simulink model "hopper_6dof"  (R2026b)
settings: Solver=FixedStepAuto  StopTime=tgrid(end)  FixedStep=1e-3  RelTol=1e-5
undefined symbols (not defined in the file): cg_init, controller_start_time, fdir_params, fsw_latency, fsw_period, g, IN, K1flat, K1flat_lo, K2grid, Klqi, nav_dt, nav_g, nav_init, nav_Qc, nav_reset, OUT, p, sensor_params, Target_Trajectory, tgrid, u_hold_command, unom, VEH
libraries: fl_lib x43, nesl_utility x31, SimscapeFluids_lib x13, slpidlib x3, simulink_extras x2, commrandsrc3 x1, dspsrcs4 x1, matrix_library x1, aerolibutil x1
(part 1 of 6)
settings Model: DataDictionary=hopper_harness.sldd  Creator=asing  LastModifiedBy=asing
settings DebuggingCC: SignalInfNanChecking=warning
settings SimscapeCC: SimscapeUseEnergyAccounting=off

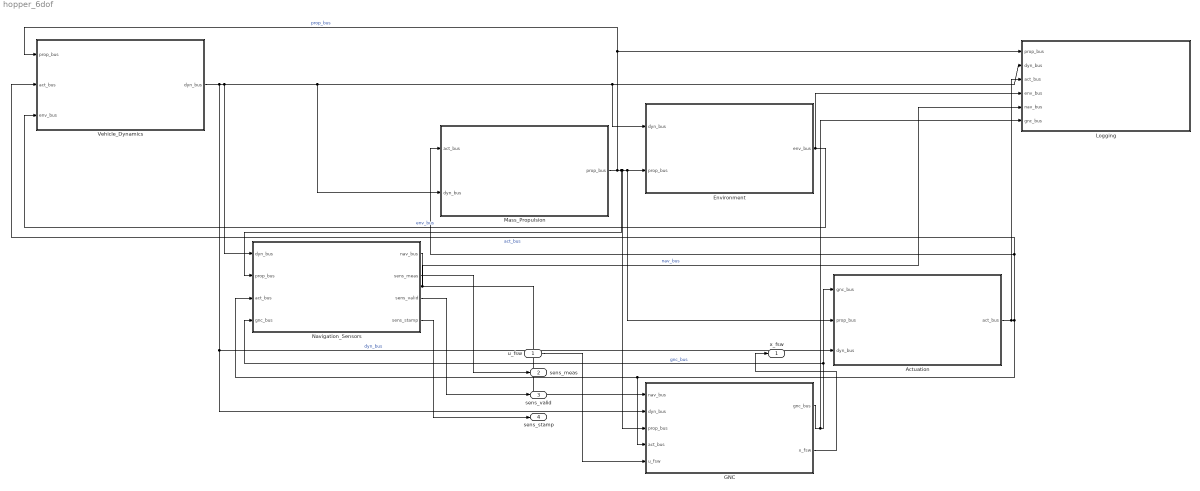
== system hopper_6dof ==
  u_fsw : Inport  OutDataTypeStr=double  PortDimensions=4  Interpolate=off
  Actuation : Subsystem
  Environment : Subsystem
  GNC : Subsystem
  Logging : Subsystem
  Mass_Propulsion : Subsystem
  Navigation_Sensors : Subsystem
  Vehicle_Dynamics : Subsystem
  x_fsw : Outport
  sens_meas : Outport  Port=2
  sens_valid : Outport  Port=3
  sens_stamp : Outport  Port=4
  wires:
  Vehicle_Dynamics/1(dyn_bus) -> GNC/2(dyn_bus), Actuation/3(dyn_bus), Environment/1(dyn_bus), Logging/2(dyn_bus), Mass_Propulsion/2(dyn_bus), Navigation_Sensors/1(dyn_bus)  "dyn_bus"
  GNC/1(gnc_bus) -> Navigation_Sensors/4(gnc_bus), Actuation/1(gnc_bus), Logging/6(gnc_bus)  "gnc_bus"
  Navigation_Sensors/1(nav_bus) -> GNC/1(nav_bus), Logging/5(nav_bus)  "nav_bus"
  Environment/1(env_bus) -> Vehicle_Dynamics/3(env_bus), Logging/4(env_bus)  "env_bus"
  Mass_Propulsion/1(prop_bus) -> Actuation/2(prop_bus), Environment/2(prop_bus), GNC/3(prop_bus), Navigation_Sensors/2(prop_bus), Logging/1(prop_bus), Vehicle_Dynamics/1(prop_bus)  "prop_bus"
  Actuation/1(act_bus) -> GNC/4(act_bus), Navigation_Sensors/3(act_bus), Mass_Propulsion/1(act_bus), Vehicle_Dynamics/2(act_bus), Logging/3(act_bus)  "act_bus"
  u_fsw/1 -> GNC/5(u_fsw)
  GNC/2(x_fsw) -> x_fsw/1
  Navigation_Sensors/2(sens_meas) -> sens_meas/1
  Navigation_Sensors/3(sens_valid) -> sens_valid/1
  Navigation_Sensors/4(sens_stamp) -> sens_stamp/1

== system hopper_6dof/Actuation ==
  u_cmd : Inport  PortName=gnc_bus  Element=u_cmd
  thrust : Inport  Port=2  PortName=prop_bus  Element=thrust
  cg : Inport  Port=2  PortName=prop_bus  Element=cg
  engine_cg : Inport  Port=2  PortName=prop_bus  Element=engine_cg
  mass : Inport  Port=2  PortName=prop_bus  Element=mass
  g_body : Inport  Port=3  PortName=dyn_bus  Element=g_body
  Actuators_TVC_RCS : Subsystem  ReferencedSubsystem=Actuators_TVC_RCS
  Demux : Demux
  IC : InitialCondition  Value=VEH.mass.wet*g
  Product : Product
  Quantizer : Quantizer  QuantizationInterval=IN.throttle_valve.resolution
  Rate Limiter1 : RateLimiter  RisingSlewLimit=IN.throttle_valve.rate_limit  FallingSlewLimit=-IN.throttle_valve.rate_limit  SampleTimeMode=inherited
  Saturation2 : Saturate  UpperLimit=IN.propulsion.nominal_thrust * IN.propulsion.throttle_range(2)  LowerLimit=IN.propulsion.nominal_thrust * IN.propulsion.throttle_range(1)
  Transport Delay2 : TransportDelay  DelayTime=IN.throttle_valve_latency
  Warmup_Control_Gate : Subsystem
  force : Outport  PortName=act_bus  Element=force
  moment : Outport  PortName=act_bus  Element=moment
  tvc_pitch : Outport  PortName=act_bus  Element=tvc_pitch
  tvc_yaw : Outport  PortName=act_bus  Element=tvc_yaw
  thrust_req : Outport  PortName=act_bus  Element=thrust_req
  thrust_cmd : Outport  PortName=act_bus  Element=thrust_cmd
  wires:
  IC/1 -> thrust_req/1, Saturation2/1
  Product/1 -> Actuators_TVC_RCS/5
  thrust/1 -> Actuators_TVC_RCS/1
  Demux/4 -> Actuators_TVC_RCS/4
  Demux/3 -> Actuators_TVC_RCS/3
  Demux/2 -> Actuators_TVC_RCS/2
  Demux/1 -> IC/1
  cg/1 -> Actuators_TVC_RCS/6
  engine_cg/1 -> Actuators_TVC_RCS/7
  Actuators_TVC_RCS/2 -> moment/1
  g_body/1 -> Product/1
  mass/1 -> Product/2, Actuators_TVC_RCS/8
  Actuators_TVC_RCS/1 -> force/1
  Actuators_TVC_RCS/3 -> tvc_pitch/1
  Actuators_TVC_RCS/4 -> tvc_yaw/1
  u_cmd/1 -> Warmup_Control_Gate/1(In1)
  Warmup_Control_Gate/1(Out1) -> Demux/1
  Quantizer/1 -> thrust_cmd/1
  Transport Delay2/1 -> Quantizer/1
  Saturation2/1 -> Rate Limiter1/1
  Rate Limiter1/1 -> Transport Delay2/1

== system hopper_6dof/Environment ==
  vel_ned : Inport  PortName=dyn_bus  Element=vel_ned
  dcm_be : Inport  PortName=dyn_bus  Element=dcm_be
  cg : Inport  Port=2  PortName=prop_bus  Element=cg
  Bernoulli Binary Generator : commrandsrc3/Bernoulli Binary Generator  ProbabilityOfZero=0.95  SeedSource=Parameter  Seed=0  SampleTime=0.1  SamplesPerFrame=1  OutputDataType=double  SimulateUsing=Interpreted execution
  MatrixMultiply1 : Product  Multiplication=Matrix(*)
  MatrixMultiply2 : Product  Multiplication=Matrix(*)
  Product1 : Product
  Random Source : dspsrcs4/Random Source  SrcType=Gaussian  MinVal=0  MaxVal=1  MeanVal=0  VarVal=IN.vehicle.disturbance.roll_torque_var  RepMode=Specify seed  rawSeed=1  IsInherit=off  SampTime=1  SampFrame=1  OutComplex=Real  DataType=double  SimulateUsing=Interpreted execution
  Wind_Forces : Subsystem  ReferencedSubsystem=Wind_Forces
  wind_force : Outport  PortName=env_bus  Element=wind_force
  wind_moment : Outport  PortName=env_bus  Element=wind_moment
  roll_dist : Outport  PortName=env_bus  Element=roll_dist
  wires:
  Bernoulli Binary Generator/1 -> Product1/1
  Random Source/1 -> Product1/2
  Wind_Forces/1 -> MatrixMultiply1/2
  Wind_Forces/2 -> MatrixMultiply2/2
  Product1/1 -> roll_dist/1
  cg/1 -> Wind_Forces/2
  vel_ned/1 -> Wind_Forces/1
  dcm_be/1 -> MatrixMultiply1/1, MatrixMultiply2/1, Wind_Forces/3
  MatrixMultiply1/1 -> wind_force/1
  MatrixMultiply2/1 -> wind_moment/1

== system hopper_6dof/GNC ==
  x_nav : Inport  PortName=nav_bus  Element=x_nav
  dcm_nav : Inport  PortName=nav_bus  Element=dcm_nav
  meas : Inport  PortName=nav_bus  Element=meas
  valid : Inport  PortName=nav_bus  Element=valid
  stamp : Inport  PortName=nav_bus  Element=stamp
  x_filt : Inport  PortName=nav_bus  Element=x_filt
  p_cov : Inport  PortName=nav_bus  Element=p_cov
  nav_diag : Inport  PortName=nav_bus  Element=nav_diag
  shadow : Inport  PortName=nav_bus  Element=shadow
  x_vert : Inport  PortName=nav_bus  Element=x_vert
  f_body : Inport  Port=2  PortName=dyn_bus  Element=f_body
  thrust : Inport  Port=3  PortName=prop_bus  Element=thrust
  mass : Inport  Port=3  PortName=prop_bus  Element=mass
  tvc_pitch : Inport  Port=4  PortName=act_bus  Element=tvc_pitch
  tvc_yaw : Inport  Port=4  PortName=act_bus  Element=tvc_yaw
  moment : Inport  Port=4  PortName=act_bus  Element=moment
  u_fsw : Inport  Port=5
  Actuator_Faults : Subsystem  Variant=on
  Controller : Subsystem  Variant=on  PropagateVariantConditions=on
  FDIR : Subsystem  Variant=on
  nav_mask : Outport  PortName=gnc_bus  Element=nav_mask
  nav_r_scale : Outport  PortName=gnc_bus  Element=nav_r_scale
  u_cmd : Outport  PortName=gnc_bus  Element=u_cmd
  x_fsw : Outport  Port=2
  wires:
  tvc_yaw/1 -> FDIR/7(tvc_yaw)
  x_nav/1 -> FDIR/2(x), Controller/1(x)
  f_body/1 -> FDIR/3(f_b)
  FDIR/3(nav_r_scale) -> nav_r_scale/1  "FDIR_nav_r_scale"
  Controller/1(u) -> FDIR/1(u_nom)
  dcm_nav/1 -> FDIR/4(dcm_be)
  meas/1 -> FDIR/10(meas)
  thrust/1 -> FDIR/5(thrust)
  tvc_pitch/1 -> FDIR/6(tvc_pitch)
  moment/1 -> FDIR/8(Mxyz)
  mass/1 -> FDIR/9(mass)
  valid/1 -> FDIR/11(valid)
  stamp/1 -> FDIR/12(stamp)
  x_filt/1 -> FDIR/13(xn)
  p_cov/1 -> FDIR/14(P)
  nav_diag/1 -> FDIR/15(diag)
  shadow/1 -> FDIR/16(shadow)
  x_vert/1 -> FDIR/17(x_vert)
  FDIR/2(nav_mask) -> nav_mask/1  "FDIR_nav_mask"
  FDIR/1(u) -> Actuator_Faults/1(u_in)
  Actuator_Faults/1(u) -> u_cmd/1
  u_fsw/1 -> Controller/2(u_fsw)
  Controller/2(x_fsw) -> x_fsw/1

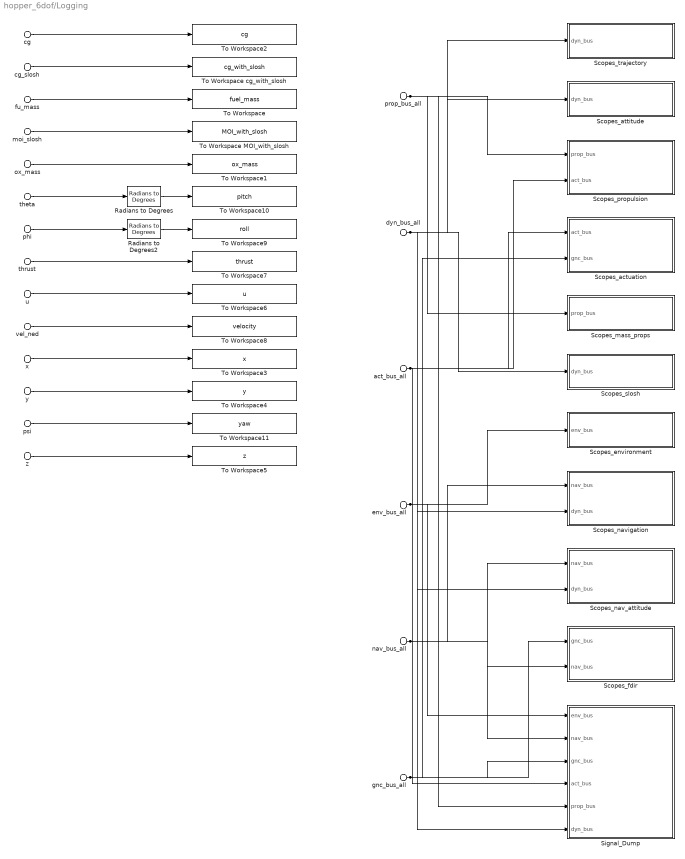
== system hopper_6dof/Logging ==
  prop_bus_all : Inport  PortName=prop_bus
  fu_mass : Inport  PortName=prop_bus  Element=fu_mass
  ox_mass : Inport  PortName=prop_bus  Element=ox_mass
  cg : Inport  PortName=prop_bus  Element=cg
  thrust : Inport  PortName=prop_bus  Element=thrust
  moi_slosh : Inport  PortName=prop_bus  Element=moi_slosh
  cg_slosh : Inport  PortName=prop_bus  Element=cg_slosh
  dyn_bus_all : Inport  Port=2  PortName=dyn_bus
  x : Inport  Port=2  PortName=dyn_bus  Element=x
  y : Inport  Port=2  PortName=dyn_bus  Element=y
  z : Inport  Port=2  PortName=dyn_bus  Element=z
  u : Inport  Port=2  PortName=dyn_bus  Element=u
  vel_ned : Inport  Port=2  PortName=dyn_bus  Element=vel_ned
  psi : Inport  Port=2  PortName=dyn_bus  Element=psi
  theta : Inport  Port=2  PortName=dyn_bus  Element=theta
  phi : Inport  Port=2  PortName=dyn_bus  Element=phi
  act_bus_all : Inport  Port=3  PortName=act_bus
  env_bus_all : Inport  Port=4  PortName=env_bus
  nav_bus_all : Inport  Port=5  PortName=nav_bus
  gnc_bus_all : Inport  Port=6  PortName=gnc_bus
  Radians to Degrees : simulink_extras/Transformations/Radians to Degrees
  Radians to Degrees2 : simulink_extras/Transformations/Radians to Degrees
  Scopes_actuation : Subsystem  Variant=on  EmptyChoice=on
  Scopes_attitude : Subsystem  Variant=on  EmptyChoice=on
  Scopes_environment : Subsystem  Variant=on  EmptyChoice=on
  Scopes_fdir : Subsystem  Variant=on  EmptyChoice=on
  Scopes_mass_props : Subsystem  Variant=on  EmptyChoice=on
  Scopes_nav_attitude : Subsystem  Variant=on  EmptyChoice=on
  Scopes_navigation : Subsystem  Variant=on  EmptyChoice=on
  Scopes_propulsion : Subsystem  Variant=on  EmptyChoice=on
  Scopes_slosh : Subsystem  Variant=on  EmptyChoice=on
  Scopes_trajectory : Subsystem  Variant=on  EmptyChoice=on
  Signal_Dump : Subsystem  Variant=on  EmptyChoice=on
  To Workspace : ToWorkspace  VariableName=fuel_mass  SaveFormat=Timeseries  SampleTime=-1
  To Workspace MOI_with_slosh : ToWorkspace  VariableName=MOI_with_slosh  SaveFormat=Timeseries  SampleTime=-1
  To Workspace cg_with_slosh : ToWorkspace  VariableName=cg_with_slosh  SaveFormat=Timeseries  SampleTime=-1
  To Workspace1 : ToWorkspace  VariableName=ox_mass  SaveFormat=Timeseries  SampleTime=-1
  To Workspace10 : ToWorkspace  VariableName=pitch  SaveFormat=Timeseries  SampleTime=-1
  To Workspace11 : ToWorkspace  VariableName=yaw  SaveFormat=Timeseries  SampleTime=-1
  To Workspace2 : ToWorkspace  VariableName=cg  SaveFormat=Timeseries  SampleTime=-1
  To Workspace3 : ToWorkspace  VariableName=x  SaveFormat=Timeseries  SampleTime=-1
  To Workspace4 : ToWorkspace  VariableName=y  SaveFormat=Timeseries  SampleTime=-1
  To Workspace5 : ToWorkspace  VariableName=z  SaveFormat=Timeseries  SampleTime=-1
  To Workspace6 : ToWorkspace  VariableName=u  SaveFormat=Timeseries  SampleTime=-1
  To Workspace7 : ToWorkspace  VariableName=thrust  SaveFormat=Timeseries  SampleTime=-1
  To Workspace8 : ToWorkspace  VariableName=velocity  SaveFormat=Timeseries  SampleTime=-1
  To Workspace9 : ToWorkspace  VariableName=roll  SaveFormat=Timeseries  SampleTime=-1
  wires:
  u/1 -> To Workspace6/1
  vel_ned/1 -> To Workspace8/1
  thrust/1 -> To Workspace7/1
  phi/1 -> Radians to Degrees2/1
  moi_slosh/1 -> To Workspace MOI_with_slosh/1
  cg_slosh/1 -> To Workspace cg_with_slosh/1
  cg/1 -> To Workspace2/1
  theta/1 -> Radians to Degrees/1
  psi/1 -> To Workspace11/1
  Radians to Degrees2/1 -> To Workspace9/1
  ox_mass/1 -> To Workspace1/1
  fu_mass/1 -> To Workspace/1
  Radians to Degrees/1 -> To Workspace10/1
  x/1 -> To Workspace3/1
  y/1 -> To Workspace4/1
  z/1 -> To Workspace5/1
  dyn_bus_all/1 -> Scopes_trajectory/1(dyn_bus), Scopes_attitude/1(dyn_bus), Scopes_slosh/1(dyn_bus), Scopes_navigation/2(dyn_bus), Scopes_nav_attitude/2(dyn_bus), Signal_Dump/6(dyn_bus)
  prop_bus_all/1 -> Scopes_propulsion/1(prop_bus), Scopes_mass_props/1(prop_bus), Signal_Dump/5(prop_bus)
  act_bus_all/1 -> Scopes_propulsion/2(act_bus), Scopes_actuation/1(act_bus), Signal_Dump/4(act_bus)
  gnc_bus_all/1 -> Scopes_actuation/2(gnc_bus), Scopes_fdir/1(gnc_bus), Signal_Dump/3(gnc_bus)
  env_bus_all/1 -> Scopes_environment/1(env_bus), Signal_Dump/1(env_bus)
  nav_bus_all/1 -> Scopes_navigation/1(nav_bus), Scopes_nav_attitude/1(nav_bus), Scopes_fdir/2(nav_bus), Signal_Dump/2(nav_bus)

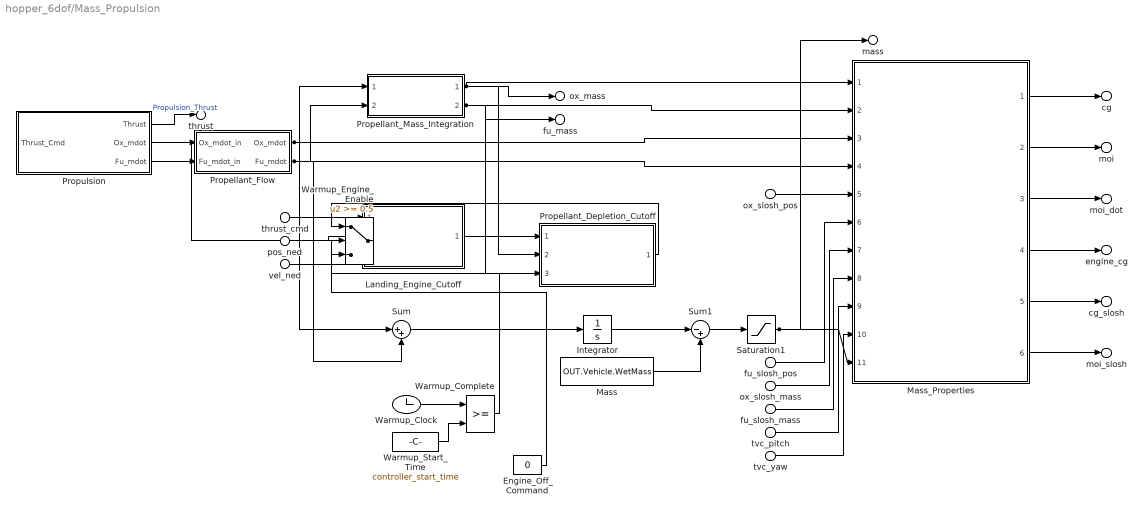
== system hopper_6dof/Mass_Propulsion ==
  thrust_cmd : Inport  PortName=act_bus  Element=thrust_cmd
  tvc_pitch : Inport  PortName=act_bus  Element=tvc_pitch
  tvc_yaw : Inport  PortName=act_bus  Element=tvc_yaw
  pos_ned : Inport  Port=2  PortName=dyn_bus  Element=pos_ned
  vel_ned : Inport  Port=2  PortName=dyn_bus  Element=vel_ned
  ox_slosh_pos : Inport  Port=2  PortName=dyn_bus  Element=ox_slosh_pos
  fu_slosh_pos : Inport  Port=2  PortName=dyn_bus  Element=fu_slosh_pos
  ox_slosh_mass : Inport  Port=2  PortName=dyn_bus  Element=ox_slosh_mass
  fu_slosh_mass : Inport  Port=2  PortName=dyn_bus  Element=fu_slosh_mass
  Engine_Off_Command : Constant  Value=0
  Integrator : Integrator
  Landing_Engine_Cutoff : Subsystem  ReferencedSubsystem=Landing_Engine_Cutoff
  Mass : Constant  Value=OUT.Vehicle.WetMass
  Mass_Properties : Subsystem  ReferencedSubsystem=Mass_Properties
  Propellant_Depletion_Cutoff : Subsystem  ReferencedSubsystem=Propellant_Depletion_Cutoff
  Propellant_Flow : Subsystem  Variant=on
  Propellant_Mass_Integration : Subsystem  ReferencedSubsystem=Propellant_Mass_Integration
  Propulsion : Subsystem  Variant=on
  Saturation1 : Saturate  UpperLimit=OUT.Vehicle.WetMass  LowerLimit=OUT.Vehicle.DryMass
  Sum : Sum  Inputs=|++
  Sum1 : Sum  Inputs=|-+
  Warmup_Clock : Clock
  Warmup_Complete : RelationalOperator  OutDataTypeStr=boolean  RndMeth=Simplest  InputSameDT=off
  Warmup_Engine_Enable : Switch  Threshold=0.5  SaturateOnIntegerOverflow=off  InputSameDT=off
  Warmup_Start_Time : Constant  Value=controller_start_time
  thrust : Outport  PortName=prop_bus  Element=thrust
  ox_mass : Outport  PortName=prop_bus  Element=ox_mass
  fu_mass : Outport  PortName=prop_bus  Element=fu_mass
  cg : Outport  PortName=prop_bus  Element=cg
  moi : Outport  PortName=prop_bus  Element=moi
  moi_dot : Outport  PortName=prop_bus  Element=moi_dot
  engine_cg : Outport  PortName=prop_bus  Element=engine_cg
  cg_slosh : Outport  PortName=prop_bus  Element=cg_slosh
  moi_slosh : Outport  PortName=prop_bus  Element=moi_slosh
  mass : Outport  PortName=prop_bus  Element=mass
  wires:
  Propulsion/1(Thrust) -> thrust/1  "Propulsion_Thrust"
  Propulsion/3(Fu_mdot) -> Propellant_Flow/2(Fu_mdot_in)
  Propellant_Mass_Integration/2 -> Mass_Properties/2, Propellant_Depletion_Cutoff/3, fu_mass/1
  Propellant_Mass_Integration/1 -> Mass_Properties/1, Propellant_Depletion_Cutoff/2, ox_mass/1
  Propulsion/2(Ox_mdot) -> Propellant_Flow/1(Ox_mdot_in)
  tvc_pitch/1 -> Mass_Properties/9
  ox_slosh_mass/1 -> Mass_Properties/7
  Propellant_Flow/1(Ox_mdot) -> Propellant_Mass_Integration/1, Mass_Properties/3, Sum/1
  Propellant_Flow/2(Fu_mdot) -> Sum/2, Mass_Properties/4, Propellant_Mass_Integration/2
  Mass_Properties/4 -> engine_cg/1
  Mass_Properties/3 -> moi_dot/1
  vel_ned/1 -> Landing_Engine_Cutoff/3
  pos_ned/1 -> Landing_Engine_Cutoff/2
  thrust_cmd/1 -> Landing_Engine_Cutoff/1
  Landing_Engine_Cutoff/1 -> Propellant_Depletion_Cutoff/1
  Sum/1 -> Integrator/1
  Integrator/1 -> Sum1/1
  Mass/1 -> Sum1/2
  Sum1/1 -> Saturation1/1
  ox_slosh_pos/1 -> Mass_Properties/5
  Saturation1/1 -> Mass_Properties/11, mass/1
  fu_slosh_pos/1 -> Mass_Properties/6
  tvc_yaw/1 -> Mass_Properties/10
  fu_slosh_mass/1 -> Mass_Properties/8
  Mass_Properties/2 -> moi/1
  Mass_Properties/1 -> cg/1
  Mass_Properties/6 -> moi_slosh/1
  Mass_Properties/5 -> cg_slosh/1
  Warmup_Clock/1 -> Warmup_Complete/1
  Warmup_Start_Time/1 -> Warmup_Complete/2
  Propellant_Depletion_Cutoff/1 -> Warmup_Engine_Enable/1
  Warmup_Complete/1 -> Warmup_Engine_Enable/2
  Engine_Off_Command/1 -> Warmup_Engine_Enable/3
  Warmup_Engine_Enable/1 -> Propulsion/1(Thrust_Cmd)

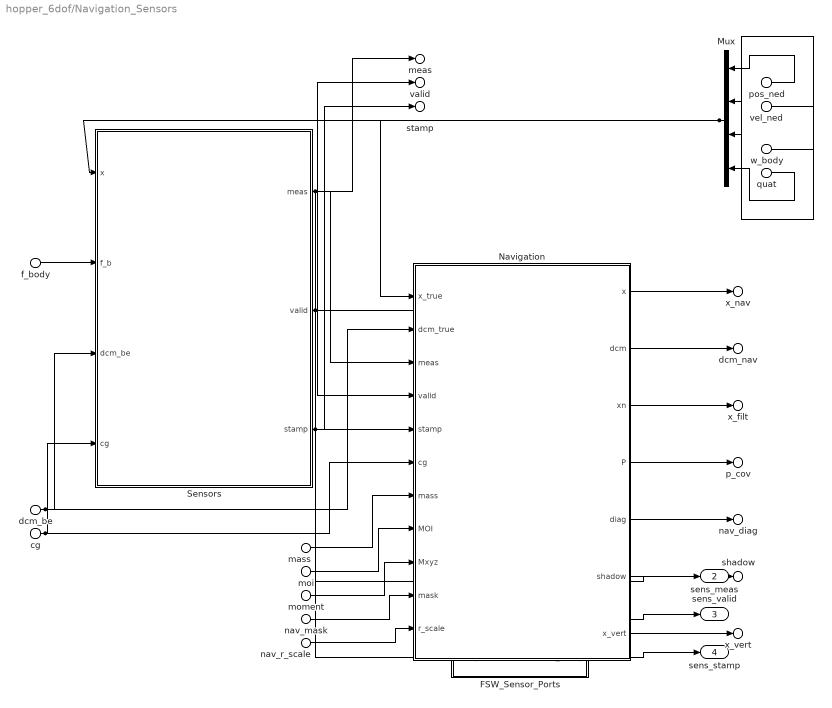
== system hopper_6dof/Navigation_Sensors ==
  f_body : Inport  PortName=dyn_bus  Element=f_body
  dcm_be : Inport  PortName=dyn_bus  Element=dcm_be
  pos_ned : Inport  PortName=dyn_bus  Element=pos_ned
  vel_ned : Inport  PortName=dyn_bus  Element=vel_ned
  w_body : Inport  PortName=dyn_bus  Element=w_body
  quat : Inport  PortName=dyn_bus  Element=quat
  cg : Inport  Port=2  PortName=prop_bus  Element=cg
  mass : Inport  Port=2  PortName=prop_bus  Element=mass
  moi : Inport  Port=2  PortName=prop_bus  Element=moi
  moment : Inport  Port=3  PortName=act_bus  Element=moment
  nav_mask : Inport  Port=4  PortName=gnc_bus  Element=nav_mask
  nav_r_scale : Inport  Port=4  PortName=gnc_bus  Element=nav_r_scale
  FSW_Sensor_Ports : Subsystem  Description=CONTROLLER=fsw only: the sensor model's meas/valid/stamp out to root sens_* ports for the flight-software plant. Built by tools/refactor/addFswSensorPorts.m.  Variant=on  EmptyChoice=on  PropagateVariantConditions=on
  Mux : Mux
  Navigation : Subsystem  Variant=on
  Sensors : Subsystem  Variant=on
  meas : Outport  PortName=nav_bus  Element=meas
  valid : Outport  PortName=nav_bus  Element=valid
  stamp : Outport  PortName=nav_bus  Element=stamp
  x_nav : Outport  PortName=nav_bus  Element=x_nav
  dcm_nav : Outport  PortName=nav_bus  Element=dcm_nav
  x_filt : Outport  PortName=nav_bus  Element=x_filt
  p_cov : Outport  PortName=nav_bus  Element=p_cov
  nav_diag : Outport  PortName=nav_bus  Element=nav_diag
  shadow : Outport  PortName=nav_bus  Element=shadow
  x_vert : Outport  PortName=nav_bus  Element=x_vert
  sens_meas : Outport  Port=2
  sens_valid : Outport  Port=3
  sens_stamp : Outport  Port=4
  wires:
  cg/1 -> Navigation/6(cg), Sensors/4(cg)
  f_body/1 -> Sensors/2(f_b)
  dcm_be/1 -> Navigation/2(dcm_true), Sensors/3(dcm_be)
  Navigation/2(dcm) -> dcm_nav/1
  Navigation/1(x) -> x_nav/1
  Sensors/1(meas) -> Navigation/3(meas), meas/1, FSW_Sensor_Ports/1(meas)
  Sensors/2(valid) -> valid/1, Navigation/4(valid), FSW_Sensor_Ports/2(valid)
  Sensors/3(stamp) -> Navigation/5(stamp), stamp/1, FSW_Sensor_Ports/3(stamp)
  mass/1 -> Navigation/7(mass)
  moi/1 -> Navigation/8(MOI)
  moment/1 -> Navigation/9(Mxyz)
  nav_mask/1 -> Navigation/10(mask)
  nav_r_scale/1 -> Navigation/11(r_scale)
  Navigation/4(P) -> p_cov/1
  Navigation/3(xn) -> x_filt/1
  vel_ned/1 -> Mux/2
  Navigation/6(shadow) -> shadow/1
  Navigation/5(diag) -> nav_diag/1
  Navigation/7(x_vert) -> x_vert/1
  Mux/1 -> Sensors/1(x), Navigation/1(x_true)
  pos_ned/1 -> Mux/1
  w_body/1 -> Mux/3
  quat/1 -> Mux/4
  FSW_Sensor_Ports/1(sens_meas) -> sens_meas/1
  FSW_Sensor_Ports/2(sens_valid) -> sens_valid/1
  FSW_Sensor_Ports/3(sens_stamp) -> sens_stamp/1

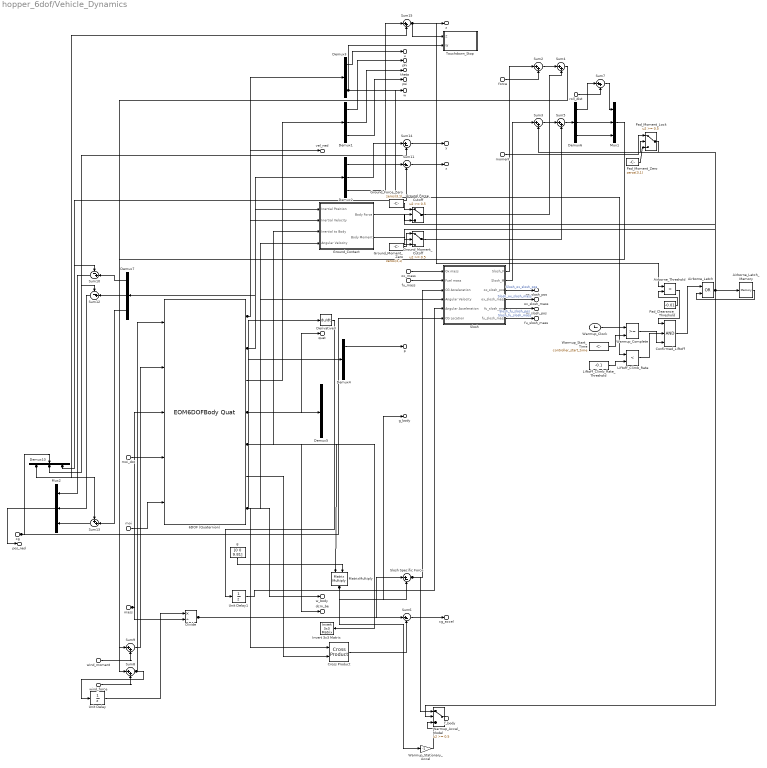
== system hopper_6dof/Vehicle_Dynamics ==
  mass : Inport  PortName=prop_bus  Element=mass
  moi_dot : Inport  PortName=prop_bus  Element=moi_dot
  moi : Inport  PortName=prop_bus  Element=moi
  ox_mass : Inport  PortName=prop_bus  Element=ox_mass
  fu_mass : Inport  PortName=prop_bus  Element=fu_mass
  cg : Inport  PortName=prop_bus  Element=cg
  force : Inport  Port=2  PortName=act_bus  Element=force
  moment : Inport  Port=2  PortName=act_bus  Element=moment
  roll_dist : Inport  Port=3  PortName=env_bus  Element=roll_dist
  wind_force : Inport  Port=3  PortName=env_bus  Element=wind_force
  wind_moment : Inport  Port=3  PortName=env_bus  Element=wind_moment
  6DOF (Quaternion) : EOM6DOFBodyQuat  mtype=Custom Variable  xme_0=[0 0 -cg_init]  eul_0=[0 pi/2 0]
  Airborne_Latch : Logic  Operator=OR  AllPortsSameDT=off  OutDataTypeStr=boolean
  Airborne_Latch_Memory : Memory
  Airborne_Threshold : RelationalOperator  Operator=<  OutDataTypeStr=boolean  RndMeth=Simplest  InputSameDT=off
  Confirmed_Liftoff : Logic  Inputs=3  AllPortsSameDT=off  OutDataTypeStr=boolean
  Cross Product : matrix_library/Cross Product
  Demux{1..4,6..7,10} (7 alike) : Demux  Outputs=3
  Demux5 : Demux
  Derivative3 : Derivative  CoefficientInTFapproximation=3
  Divide : Product  Inputs=*/
  Ground_Contact : Subsystem  Variant=on
  Ground_Force_Cutoff : Switch  Threshold=0.5  SaturateOnIntegerOverflow=off  InputSameDT=off
  Ground_Force_Zero : Constant  Value=zeros(3,1)
  Ground_Moment_Cutoff : Switch  Threshold=0.5  SaturateOnIntegerOverflow=off  InputSameDT=off
  Ground_Moment_Zero : Constant  Value=zeros(3,1)
  Invert 3x3 Matrix : aerolibutil/Invert  3x3 Matrix
  Liftoff_Climb_Rate : RelationalOperator  Operator=<  OutDataTypeStr=boolean  RndMeth=Simplest  InputSameDT=off
  Liftoff_Climb_Rate_Threshold : Constant  Value=-0.1
  MatrixMultiply : Product  Multiplication=Matrix(*)
  Mux1 : Mux  Inputs=3
  Mux2 : Mux  Inputs=3
  Pad_Clearance_Threshold : Constant  Value=-0.01
  Pad_Moment_Lock : Switch  Threshold=0.5  SaturateOnIntegerOverflow=off  InputSameDT=off
  Pad_Moment_Zero : Constant  Value=zeros(3,1)
  Slosh : Subsystem  Variant=on
  Slosh Specific Force : Sum  Description=(F_total/m) - g_body = non-gravitational specific force at the CG; drives the slosh pendulums.  Inputs=|+-
  Sum10 : Sum  Inputs=-+|
  Sum11 : Sum  Inputs=|+-
  Sum12 : Sum  Inputs=-+|
  Sum13 : Sum  Inputs=++|
  Sum14 : Sum  Inputs=|+-
  Sum{2..5,7..9,15} (8 alike) : Sum  Inputs=|++
  Sum6 : Sum  Inputs=|+-
  Touchdown_Stop : Subsystem  Description=Stops the run at the first descending ground contact, except with CONTROLLER=fsw and GROUND=strut (the flight software's plant rests on its struts). Built by tools/refactor/gateTouchdownStop.m.  Variant=on  EmptyChoice=on
  Unit Delay : UnitDelay  SampleTime=-1
  Unit Delay1 : UnitDelay  SampleTime=-1
  Warmup_Accel_Model : Switch  Threshold=0.5  SaturateOnIntegerOverflow=off  InputSameDT=off
  Warmup_Clock : Clock
  Warmup_Complete : RelationalOperator  OutDataTypeStr=boolean  RndMeth=Simplest  InputSameDT=off
  Warmup_Start_Time : Constant  Value=controller_start_time
  Warmup_Stationary_Accel : Gain  Gain=-1
  g : Constant  Value=[0 0 9.81]
  vel_ned : Outport  PortName=dyn_bus  Element=vel_ned
  quat : Outport  PortName=dyn_bus  Element=quat
  dcm_be : Outport  PortName=dyn_bus  Element=dcm_be
  w_body : Outport  PortName=dyn_bus  Element=w_body
  ox_slosh_pos : Outport  PortName=dyn_bus  Element=ox_slosh_pos
  ox_slosh_mass : Outport  PortName=dyn_bus  Element=ox_slosh_mass
  fu_slosh_pos : Outport  PortName=dyn_bus  Element=fu_slosh_pos
  fu_slosh_mass : Outport  PortName=dyn_bus  Element=fu_slosh_mass
  f_body : Outport  PortName=dyn_bus  Element=f_body
  cg_accel : Outport  PortName=dyn_bus  Element=cg_accel
  x : Outport  PortName=dyn_bus  Element=x
  y : Outport  PortName=dyn_bus  Element=y
  z : Outport  PortName=dyn_bus  Element=z
  phi : Outport  PortName=dyn_bus  Element=phi
  theta : Outport  PortName=dyn_bus  Element=theta
  psi : Outport  PortName=dyn_bus  Element=psi
  u : Outport  PortName=dyn_bus  Element=u
  w : Outport  PortName=dyn_bus  Element=w
  p : Outport  PortName=dyn_bus  Element=p
  pos_ned : Outport  PortName=dyn_bus  Element=pos_ned
  g_body : Outport  PortName=dyn_bus  Element=g_body
  wires:
  cg/1 -> Demux10/1, Slosh/6(CG Location)
  Sum13/1 -> Mux2/3
  Demux10/3 -> Sum10/1, Sum11/2
  Demux10/2 -> Sum12/1, Sum14/2
  Demux10/1 -> Sum13/1, Sum15/2
  Mux2/1 -> pos_ned/1
  MatrixMultiply/1 -> Slosh Specific Force/2, g_body/1, Warmup_Stationary_Accel/1
  Sum10/1 -> Mux2/1
  Sum12/1 -> Mux2/2
  wind_moment/1 -> Sum9/2
  wind_force/1 -> Sum8/2
  Unit Delay/1 -> Divide/1
  Demux7/3 -> Sum13/2
  Demux7/1 -> Sum10/2
  Demux7/2 -> Sum12/2
  moi_dot/1 -> 6DOF (Quaternion)/4
  moi/1 -> 6DOF (Quaternion)/5
  mass/1 -> 6DOF (Quaternion)/3, Divide/2
  Derivative3/1 -> Unit Delay1/1
  Sum9/1 -> 6DOF (Quaternion)/2
  Sum8/1 -> Unit Delay/1, 6DOF (Quaternion)/1
  g/1 -> MatrixMultiply/2
  Demux1/3 -> psi/1
  Demux1/2 -> theta/1
  6DOF (Quaternion)/1 -> Ground_Contact/2(Inertial Velocity), Demux3/1, vel_ned/1
  Unit Delay1/1 -> Slosh/5(Angular Acceleration)
  6DOF (Quaternion)/2 -> Demux7/1, Ground_Contact/1(Inertial Position), Demux2/1
  6DOF (Quaternion)/3 -> Demux1/1
  6DOF (Quaternion)/4 -> quat/1, Demux5/1
  Demux6/1 -> Sum7/1
  6DOF (Quaternion)/5 -> Invert 3x3 Matrix/1, Ground_Contact/3(Inertial to Body), MatrixMultiply/1, dcm_be/1
  6DOF (Quaternion)/6 -> Cross Product/2
  6DOF (Quaternion)/7 -> Demux4/1, Slosh/4(Angular Velocity), Cross Product/1, Derivative3/1, Ground_Contact/4(Angular Velocity), w_body/1
  Divide/1 -> Slosh Specific Force/1, Sum6/1
  Demux3/1 -> u/1
  Demux3/3 -> w/1, Liftoff_Climb_Rate/1, Touchdown_Stop/2(W)
  Demux1/1 -> phi/1
  Demux2/2 -> Sum14/1
  Demux2/1 -> Sum11/1
  Demux2/3 -> Sum15/1
  Demux4/1 -> p/1
  Sum3/1 -> Sum5/1
  Slosh/1(Slosh_F) -> Sum2/1
  Cross Product/1 -> Sum6/2
  Sum15/1 -> z/1, Airborne_Threshold/1, Touchdown_Stop/1(Z)
  Sum14/1 -> y/1
  Sum11/1 -> x/1
  ox_mass/1 -> Slosh/1(Ox mass)
  fu_mass/1 -> Slosh/2(Fuel mass)
  Slosh Specific Force/1 -> Slosh/3(CG Acceleration), Warmup_Accel_Model/1
  Sum6/1 -> cg_accel/1
  force/1 -> Sum2/2
  Slosh/3(ox_slosh_pos) -> ox_slosh_pos/1  "Slosh_ox_slosh_pos"
  Slosh/2(Slosh_M) -> Sum3/1
  Sum4/1 -> Sum8/1
  Slosh/5(fu_slosh_pos) -> fu_slosh_pos/1  "Slosh_fu_slosh_pos"
  Slosh/4(ox_slosh_mass) -> ox_slosh_mass/1  "Slosh_ox_slosh_mass"
  Slosh/6(fu_slosh_mass) -> fu_slosh_mass/1  "Slosh_fu_slosh_mass"
  Sum2/1 -> Sum4/1
  roll_dist/1 -> Sum7/2
  Demux6/2 -> Mux1/2
  Demux6/3 -> Mux1/3
  Sum7/1 -> Mux1/1
  Mux1/1 -> Sum9/1
  ? -> ?
  ? -> ?
  Ground_Force_Zero/1 -> Ground_Force_Cutoff/1
  Ground_Contact/1(Body Force) -> Ground_Force_Cutoff/3
  Ground_Force_Cutoff/1 -> Sum4/2
  Ground_Moment_Zero/1 -> Ground_Moment_Cutoff/1
  Ground_Contact/2(Body Moment) -> Ground_Moment_Cutoff/3
  Ground_Moment_Cutoff/1 -> Sum5/2
  Warmup_Stationary_Accel/1 -> Warmup_Accel_Model/3
  Warmup_Accel_Model/1 -> f_body/1
  Pad_Clearance_Threshold/1 -> Airborne_Threshold/2
  Airborne_Latch_Memory/1 -> Airborne_Latch/2
  Airborne_Latch/1 -> Airborne_Latch_Memory/1, Ground_Force_Cutoff/2, Ground_Moment_Cutoff/2, Warmup_Accel_Model/2, Pad_Moment_Lock/2
  Pad_Moment_Zero/1 -> Pad_Moment_Lock/3
  Warmup_Clock/1 -> Warmup_Complete/1
  Warmup_Start_Time/1 -> Warmup_Complete/2
  Liftoff_Climb_Rate_Threshold/1 -> Liftoff_Climb_Rate/2
  Airborne_Threshold/1 -> Confirmed_Liftoff/1
  Liftoff_Climb_Rate/1 -> Confirmed_Liftoff/2
  Warmup_Complete/1 -> Confirmed_Liftoff/3
  Confirmed_Liftoff/1 -> Airborne_Latch/1
  moment/1 -> Pad_Moment_Lock/1
  Pad_Moment_Lock/1 -> Sum3/2
  Sum5/1 -> Demux6/1

== system hopper_6dof/Actuation/Warmup_Control_Gate ==
  In1 : Inport
  After_Warmup : RelationalOperator  OutDataTypeStr=boolean  RndMeth=Simplest  InputSameDT=off
  Clock : Clock
  Hold_Command : Constant  Value=u_hold_command
  Select_Command : Switch  Threshold=0.5  SaturateOnIntegerOverflow=off  InputSameDT=off
  Start_Time : Constant  Value=controller_start_time
  Out1 : Outport
  wires:
  In1/1 -> Select_Command/1
  Clock/1 -> After_Warmup/1
  Start_Time/1 -> After_Warmup/2
  After_Warmup/1 -> Select_Command/2
  Hold_Command/1 -> Select_Command/3
  Select_Command/1 -> Out1/1

== system hopper_6dof/GNC/Actuator_Faults ==
  u_in : Inport
  Actuator_Faults_Off : Subsystem  VariantControl=VARIANT_FAULT_INJECTION == 1
  Actuator_Faults_On : Subsystem  VariantControl=VARIANT_FAULT_INJECTION == 2
  u : Outport

== system hopper_6dof/GNC/Controller ==
  x : Inport
  u_fsw : Inport  Port=2
  Controller_FSW : Subsystem  VariantControl=VARIANT_CONTROLLER == 5
  Controller_LQI : Subsystem  VariantControl=VARIANT_CONTROLLER == 2
  Controller_LQR_CTV_Tuning : Subsystem  VariantControl=VARIANT_CONTROLLER == 4
  Controller_LQR_Sched : Subsystem  VariantControl=VARIANT_CONTROLLER == 1
  Controller_LQR_Sched_Legacy : Subsystem  VariantControl=VARIANT_CONTROLLER == 3
  u : Outport
  x_fsw : Outport  Port=2

== system hopper_6dof/GNC/FDIR ==
  u_nom : Inport
  x : Inport  Port=2
  f_b : Inport  Port=3
  dcm_be : Inport  Port=4
  thrust : Inport  Port=5
  tvc_pitch : Inport  Port=6
  tvc_yaw : Inport  Port=7
  Mxyz : Inport  Port=8
  mass : Inport  Port=9
  meas : Inport  Port=10
  valid : Inport  Port=11
  stamp : Inport  Port=12
  xn : Inport  Port=13
  P : Inport  Port=14
  diag : Inport  Port=15
  shadow : Inport  Port=16
  x_vert : Inport  Port=17
  FDIR_Off : Subsystem  VariantControl=VARIANT_FDIR == 1
  FDIR_On : Subsystem  VariantControl=VARIANT_FDIR == 2
  u : Outport
  nav_mask : Outport  Port=2
  nav_r_scale : Outport  Port=3

== system hopper_6dof/Logging/Scopes_actuation ==
  act_bus : Inport
  gnc_bus : Inport  Port=2
  On : Subsystem  VariantControl=VARIANT_SCOPES_ACTUATION == 2

== system hopper_6dof/Logging/Scopes_attitude ==
  dyn_bus : Inport
  On : Subsystem  VariantControl=VARIANT_SCOPES_ATTITUDE == 2

== system hopper_6dof/Logging/Scopes_environment ==
  env_bus : Inport
  On : Subsystem  VariantControl=VARIANT_SCOPES_ENVIRONMENT == 2

== system hopper_6dof/Logging/Scopes_fdir ==
  gnc_bus : Inport
  nav_bus : Inport  Port=2
  On : Subsystem  VariantControl=VARIANT_SCOPES_FDIR == 2

== system hopper_6dof/Logging/Scopes_mass_props ==
  prop_bus : Inport
  On : Subsystem  VariantControl=VARIANT_SCOPES_MASS_PROPS == 2

== system hopper_6dof/Logging/Scopes_nav_attitude ==
  nav_bus : Inport
  dyn_bus : Inport  Port=2
  On : Subsystem  VariantControl=VARIANT_SCOPES_NAV_ATTITUDE == 2

== system hopper_6dof/Logging/Scopes_navigation ==
  nav_bus : Inport
  dyn_bus : Inport  Port=2
  On : Subsystem  VariantControl=VARIANT_SCOPES_NAVIGATION == 2

== system hopper_6dof/Logging/Scopes_propulsion ==
  prop_bus : Inport
  act_bus : Inport  Port=2
  On : Subsystem  VariantControl=VARIANT_SCOPES_PROPULSION == 2

== system hopper_6dof/Logging/Scopes_slosh ==
  dyn_bus : Inport
  On : Subsystem  VariantControl=VARIANT_SCOPES_SLOSH == 2

== system hopper_6dof/Logging/Scopes_trajectory ==
  dyn_bus : Inport
  On : Subsystem  VariantControl=VARIANT_SCOPES_TRAJECTORY == 2

== system hopper_6dof/Logging/Signal_Dump ==
  env_bus : Inport
  nav_bus : Inport  Port=2
  gnc_bus : Inport  Port=3
  act_bus : Inport  Port=4
  prop_bus : Inport  Port=5
  dyn_bus : Inport  Port=6
  On : Subsystem  VariantControl=VARIANT_LOG == 2

== system hopper_6dof/Mass_Propulsion/Propellant_Flow ==
  Ox_mdot_in : Inport
  Fu_mdot_in : Inport  Port=2
  Flow_Constant : Subsystem  VariantControl=VARIANT_MASS_PROPS == 2
  Flow_Varying : Subsystem  VariantControl=VARIANT_MASS_PROPS == 1
  Ox_mdot : Outport
  Fu_mdot : Outport  Port=2

== system hopper_6dof/Mass_Propulsion/Propulsion ==
  Thrust_Cmd : Inport
  Propulsion_Fluid_Network : Subsystem  VariantControl=VARIANT_PROPULSION == 2
  Propulsion_LUT : Subsystem  VariantControl=VARIANT_PROPULSION == 1
  Thrust : Outport
  Ox_mdot : Outport  Port=2
  Fu_mdot : Outport  Port=3

== system hopper_6dof/Navigation_Sensors/FSW_Sensor_Ports ==
  note: 1) Add Subsystem or Model blocks as valid variant choices.
      | 2) You cannot connect blocks at this level. At simulation, connectivity is automatically
      | determined, based on the active variant and port name matching.
  meas : Inport
  valid : Inport  Port=2
  stamp : Inport  Port=3
  FSW_Sensor_Ports_On : Subsystem  VariantControl=VARIANT_CONTROLLER == 5
  sens_meas : Outport
  sens_valid : Outport  Port=2
  sens_stamp : Outport  Port=3

== system hopper_6dof/Navigation_Sensors/Navigation ==
  x_true : Inport
  dcm_true : Inport  Port=2
  meas : Inport  Port=3
  valid : Inport  Port=4
  stamp : Inport  Port=5
  cg : Inport  Port=6
  mass : Inport  Port=7
  MOI : Inport  Port=8
  Mxyz : Inport  Port=9
  mask : Inport  Port=10
  r_scale : Inport  Port=11
  Navigation_GMEKF : Subsystem  VariantControl=VARIANT_NAVIGATION == 3
  Navigation_None : Subsystem  VariantControl=VARIANT_NAVIGATION == 1
  Navigation_Shadow : Subsystem  VariantControl=VARIANT_NAVIGATION == 2
  x : Outport
  dcm : Outport  Port=2
  xn : Outport  Port=3
  P : Outport  Port=4
  diag : Outport  Port=5
  shadow : Outport  Port=6
  x_vert : Outport  Port=7

== system hopper_6dof/Navigation_Sensors/Sensors ==
  x : Inport
  f_b : Inport  Port=2
  dcm_be : Inport  Port=3
  cg : Inport  Port=4
  Sensors_Off : Subsystem  VariantControl=~(VARIANT_FDIR == 2 || VARIANT_NAVIGATION > 1 || VARIANT_CONTROLLER == 5)
  Sensors_On : Subsystem  VariantControl=VARIANT_FDIR == 2 || VARIANT_NAVIGATION > 1 || VARIANT_CONTROLLER == 5
  meas : Outport
  valid : Outport  Port=2
  stamp : Outport  Port=3

== system hopper_6dof/Vehicle_Dynamics/Ground_Contact ==
  Inertial Position : Inport
  Inertial Velocity : Inport  Port=2
  Inertial to Body : Inport  Port=3
  Angular Velocity : Inport  Port=4
  Ground_None : Subsystem  VariantControl=VARIANT_GROUND == 1
  Ground_Strut : Subsystem  VariantControl=VARIANT_GROUND == 2
  Body Force : Outport
  Body Moment : Outport  Port=2

== system hopper_6dof/Vehicle_Dynamics/Slosh ==
  Ox mass : Inport
  Fuel mass : Inport  Port=2
  CG Acceleration : Inport  Port=3
  Angular Velocity : Inport  Port=4
  Angular Acceleration : Inport  Port=5
  CG Location : Inport  Port=6
  Slosh_Full : Subsystem  VariantControl=VARIANT_SLOSH == 1  ReferencedSubsystem=Slosh
  Slosh_Off : Subsystem  VariantControl=VARIANT_SLOSH == 2
  Slosh_F : Outport
  Slosh_M : Outport  Port=2
  ox_slosh_pos : Outport  Port=3
  ox_slosh_mass : Outport  Port=4
  fu_slosh_pos : Outport  Port=5
  fu_slosh_mass : Outport  Port=6

== system hopper_6dof/Vehicle_Dynamics/Touchdown_Stop ==
  note: 1) Add Subsystem or Model blocks as valid variant choices.
      | 2) You cannot connect blocks at this level. At simulation, connectivity is automatically
      | determined, based on the active variant and port name matching.
  Z : Inport
  W : Inport  Port=2
  Stop : Subsystem  VariantControl=~(VARIANT_CONTROLLER == 5 && VARIANT_GROUND == 2)  ReferencedSubsystem=Touchdown_Stop

== system hopper_6dof/GNC/Actuator_Faults/Actuator_Faults_Off ==
  u_in : Inport
  u : Outport
  wires:
  u_in/1 -> u/1

== system hopper_6dof/GNC/Actuator_Faults/Actuator_Faults_On ==
  u_in : Inport
  Actuator_Gate : MATLAB Function  TreatAsAtomicUnit=on
  Actuator_Gate_State : MATLAB Function  TreatAsAtomicUnit=on  SystemSampleTime=1e-3
  Clock : Clock
  u : Outport
  wires:
  u_in/1 -> Actuator_Gate_State/1(u_in), Actuator_Gate/1(u_in)
  Clock/1 -> Actuator_Gate_State/2(t), Actuator_Gate/2(t)
  Actuator_Gate_State/1(hold) -> Actuator_Gate/3(hold)
  Actuator_Gate_State/2(slow) -> Actuator_Gate/4(slow)
  Actuator_Gate/1(u) -> u/1

== system hopper_6dof/GNC/Controller/Controller_FSW ==
  x : Inport
  u_fsw : Inport  Port=2
  FSW_Period_Hold : ZeroOrderHold  SampleTime=[fsw_period, fsw_latency]
  u : Outport
  x_fsw : Outport  Port=2
  wires:
  u_fsw/1 -> FSW_Period_Hold/1
  FSW_Period_Hold/1 -> u/1
  x/1 -> x_fsw/1

== system hopper_6dof/GNC/Controller/Controller_LQI ==
  x : Inport
  LQI_Gain : Gain  Gain=-Klqi  Multiplication=Matrix(K*u)
  LQI_State : Mux
  MRP Correction : Subsystem
  Position : Selector  InputPortWidth=13  IndexOptions=Index vector (dialog)  Indices=1:3  OutputSizes=1  RuntimeRangeChecks=off
  Position_Command : Constant  Value=[0 0 0]
  Position_Error : Sum  Inputs=+-
  Position_Error_Integral : Integrator  InitialCondition=[0 0 0]
  Quaternion : Selector  InputPortWidth=13  IndexOptions=Index vector (dialog)  Indices=10:13  OutputSizes=1  RuntimeRangeChecks=off
  Vel_Rates : Selector  InputPortWidth=13  IndexOptions=Index vector (dialog)  Indices=4:9  OutputSizes=1  RuntimeRangeChecks=off
  q to MRP : Subsystem
  u : Outport
  wires:
  x/1 -> Position/1, Vel_Rates/1, Quaternion/1
  Quaternion/1 -> q to MRP/1(In1)
  q to MRP/1(Out1) -> MRP Correction/1(In1)
  Position/1 -> Position_Error/1
  Position_Command/1 -> Position_Error/2
  Position_Error/1 -> Position_Error_Integral/1, LQI_State/1
  Vel_Rates/1 -> LQI_State/2
  MRP Correction/1(Out1) -> LQI_State/3
  Position_Error_Integral/1 -> LQI_State/4
  LQI_State/1 -> LQI_Gain/1
  LQI_Gain/1 -> u/1

== system hopper_6dof/GNC/Controller/Controller_LQR_CTV_Tuning ==
  x : Inport
  LQR_CTV_Tuning : Subsystem  ReferencedSubsystem=LQR_CTV_Tuning
  u : Outport
  wires:
  x/1 -> LQR_CTV_Tuning/1
  LQR_CTV_Tuning/1 -> u/1

== system hopper_6dof/GNC/Controller/Controller_LQR_Sched ==
  x : Inport
  Clock : Clock
  Constant4 : Constant  Value=tgrid
  Constant5 : Constant  Value=K1flat
  Constant6 : Constant  Value=K2grid
  Constant7 : Constant  Value=unom
  Constant8 : Constant  Value=Target_Trajectory
  LQR_Gain_Scheduler : Subsystem  ReferencedSubsystem=LQR_Gain_Scheduler
  u : Outport
  wires:
  Clock/1 -> LQR_Gain_Scheduler/1
  x/1 -> LQR_Gain_Scheduler/2
  Constant4/1 -> LQR_Gain_Scheduler/3
  Constant8/1 -> LQR_Gain_Scheduler/4
  Constant5/1 -> LQR_Gain_Scheduler/5
  Constant6/1 -> LQR_Gain_Scheduler/6
  Constant7/1 -> LQR_Gain_Scheduler/7
  LQR_Gain_Scheduler/1 -> u/1

== system hopper_6dof/GNC/Controller/Controller_LQR_Sched_Legacy ==
  x : Inport
  Clock : Clock
  Constant4 : Constant  Value=tgrid
  Constant5 : Constant  Value=K1flat
  Constant6 : Constant  Value=K2grid
  Constant7 : Constant  Value=unom
  Constant8 : Constant  Value=Target_Trajectory
  Gain_Selector_Legacy : MATLAB Function  TreatAsAtomicUnit=on
  u : Outport
  wires:
  Clock/1 -> Gain_Selector_Legacy/1(t)
  x/1 -> Gain_Selector_Legacy/2(x)
  Constant4/1 -> Gain_Selector_Legacy/3(tgrid)
  Constant8/1 -> Gain_Selector_Legacy/4(xref)
  Constant5/1 -> Gain_Selector_Legacy/5(K1flat)
  Constant6/1 -> Gain_Selector_Legacy/6(K2grid)
  Constant7/1 -> Gain_Selector_Legacy/7(unom)
  Gain_Selector_Legacy/1(u) -> u/1

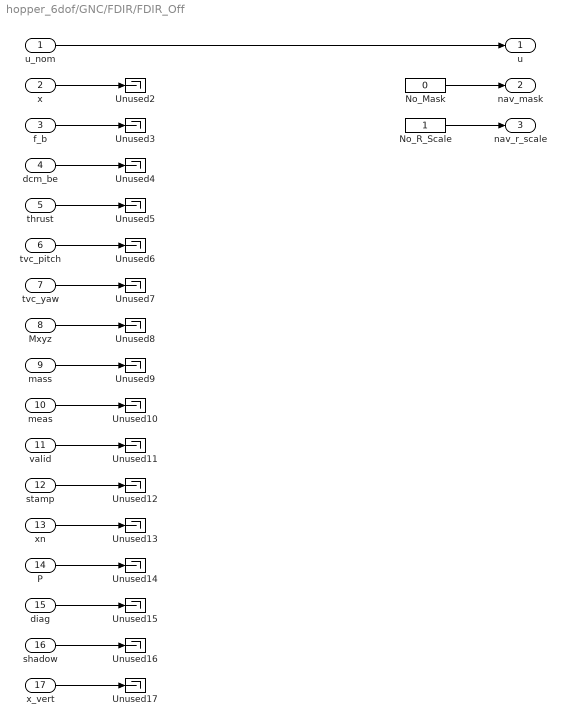
== system hopper_6dof/GNC/FDIR/FDIR_Off ==
  u_nom : Inport
  x : Inport  Port=2
  f_b : Inport  Port=3
  dcm_be : Inport  Port=4
  thrust : Inport  Port=5
  tvc_pitch : Inport  Port=6
  tvc_yaw : Inport  Port=7
  Mxyz : Inport  Port=8
  mass : Inport  Port=9
  meas : Inport  Port=10
  valid : Inport  Port=11
  stamp : Inport  Port=12
  xn : Inport  Port=13
  P : Inport  Port=14
  diag : Inport  Port=15
  shadow : Inport  Port=16
  x_vert : Inport  Port=17
  No_Mask : Constant  Value=0
  No_R_Scale : Constant
  Unused{2..17} (16 alike) : Terminator
  u : Outport
  nav_mask : Outport  Port=2
  nav_r_scale : Outport  Port=3
  wires:
  u_nom/1 -> u/1
  x/1 -> Unused2/1
  f_b/1 -> Unused3/1
  dcm_be/1 -> Unused4/1
  thrust/1 -> Unused5/1
  tvc_pitch/1 -> Unused6/1
  tvc_yaw/1 -> Unused7/1
  Mxyz/1 -> Unused8/1
  mass/1 -> Unused9/1
  meas/1 -> Unused10/1
  valid/1 -> Unused11/1
  stamp/1 -> Unused12/1
  xn/1 -> Unused13/1
  P/1 -> Unused14/1
  diag/1 -> Unused15/1
  shadow/1 -> Unused16/1
  x_vert/1 -> Unused17/1
  No_Mask/1 -> nav_mask/1
  No_R_Scale/1 -> nav_r_scale/1

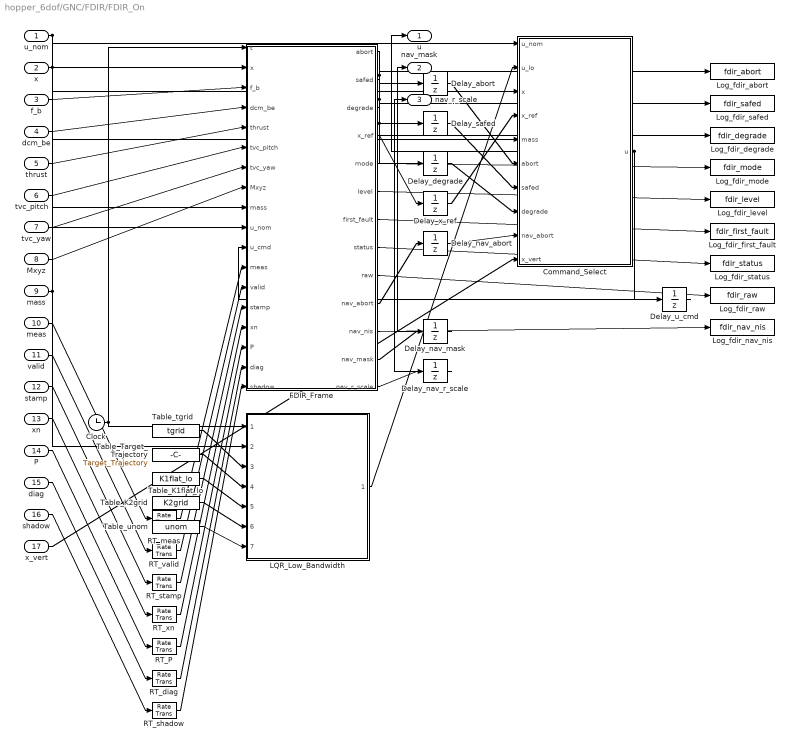
== system hopper_6dof/GNC/FDIR/FDIR_On ==
  u_nom : Inport
  x : Inport  Port=2
  f_b : Inport  Port=3
  dcm_be : Inport  Port=4
  thrust : Inport  Port=5
  tvc_pitch : Inport  Port=6
  tvc_yaw : Inport  Port=7
  Mxyz : Inport  Port=8
  mass : Inport  Port=9
  meas : Inport  Port=10
  valid : Inport  Port=11
  stamp : Inport  Port=12
  xn : Inport  Port=13
  P : Inport  Port=14
  diag : Inport  Port=15
  shadow : Inport  Port=16
  x_vert : Inport  Port=17
  Clock : Clock
  Command_Select : MATLAB Function  TreatAsAtomicUnit=on
  Delay_abort : UnitDelay  SampleTime=fdir_params.S.frame
  Delay_degrade : UnitDelay  SampleTime=fdir_params.S.frame
  Delay_nav_abort : UnitDelay  SampleTime=fdir_params.S.frame
  Delay_nav_mask : UnitDelay  SampleTime=fdir_params.S.frame
  Delay_nav_r_scale : UnitDelay  InitialCondition=1  SampleTime=fdir_params.S.frame
  Delay_safed : UnitDelay  SampleTime=fdir_params.S.frame
  Delay_u_cmd : UnitDelay  InitialCondition=zeros(4,1)  SampleTime=fdir_params.S.frame
  Delay_x_ref : UnitDelay  InitialCondition=zeros(13,1)  SampleTime=fdir_params.S.frame
  FDIR_Frame : MATLAB Function  TreatAsAtomicUnit=on  SystemSampleTime=0.01
  LQR_Low_Bandwidth : Subsystem  ReferencedSubsystem=LQR_Gain_Scheduler
  Log_fdir_abort : ToWorkspace  VariableName=fdir_abort  SaveFormat=Timeseries
  Log_fdir_degrade : ToWorkspace  VariableName=fdir_degrade  SaveFormat=Timeseries
  Log_fdir_first_fault : ToWorkspace  VariableName=fdir_first_fault  SaveFormat=Timeseries
  Log_fdir_level : ToWorkspace  VariableName=fdir_level  SaveFormat=Timeseries
  Log_fdir_mode : ToWorkspace  VariableName=fdir_mode  SaveFormat=Timeseries
  Log_fdir_nav_nis : ToWorkspace  VariableName=fdir_nav_nis  SaveFormat=Timeseries
  Log_fdir_raw : ToWorkspace  VariableName=fdir_raw  SaveFormat=Timeseries
  Log_fdir_safed : ToWorkspace  VariableName=fdir_safed  SaveFormat=Timeseries
  Log_fdir_status : ToWorkspace  VariableName=fdir_status  SaveFormat=Timeseries
  RT_P : RateTransition  OutPortSampleTime=fdir_params.S.frame
  RT_diag : RateTransition  OutPortSampleTime=fdir_params.S.frame
  RT_meas : RateTransition  OutPortSampleTime=fdir_params.S.frame
  RT_shadow : RateTransition  OutPortSampleTime=fdir_params.S.frame
  RT_stamp : RateTransition  OutPortSampleTime=fdir_params.S.frame
  RT_valid : RateTransition  OutPortSampleTime=fdir_params.S.frame
  RT_xn : RateTransition  OutPortSampleTime=fdir_params.S.frame
  Table_K1flat_lo : Constant  Value=K1flat_lo
  Table_K2grid : Constant  Value=K2grid
  Table_Target_Trajectory : Constant  Value=Target_Trajectory
  Table_tgrid : Constant  Value=tgrid
  Table_unom : Constant  Value=unom
  u : Outport
  nav_mask : Outport  Port=2
  nav_r_scale : Outport  Port=3
  wires:
  meas/1 -> RT_meas/1
  valid/1 -> RT_valid/1
  stamp/1 -> RT_stamp/1
  xn/1 -> RT_xn/1
  P/1 -> RT_P/1
  diag/1 -> RT_diag/1
  shadow/1 -> RT_shadow/1
  Clock/1 -> FDIR_Frame/1(t), LQR_Low_Bandwidth/1
  x/1 -> FDIR_Frame/2(x), LQR_Low_Bandwidth/2, Command_Select/3(x)
  f_b/1 -> FDIR_Frame/3(f_b)
  dcm_be/1 -> FDIR_Frame/4(dcm_be)
  thrust/1 -> FDIR_Frame/5(thrust)
  tvc_pitch/1 -> FDIR_Frame/6(tvc_pitch)
  tvc_yaw/1 -> FDIR_Frame/7(tvc_yaw)
  Mxyz/1 -> FDIR_Frame/8(Mxyz)
  mass/1 -> FDIR_Frame/9(mass), Command_Select/5(mass)
  u_nom/1 -> FDIR_Frame/10(u_nom), Command_Select/1(u_nom)
  RT_meas/1 -> FDIR_Frame/12(meas)
  RT_valid/1 -> FDIR_Frame/13(valid)
  RT_stamp/1 -> FDIR_Frame/14(stamp)
  RT_xn/1 -> FDIR_Frame/15(xn)
  RT_P/1 -> FDIR_Frame/16(P)
  RT_diag/1 -> FDIR_Frame/17(diag)
  RT_shadow/1 -> FDIR_Frame/18(shadow)
  FDIR_Frame/12(nav_mask) -> Delay_nav_mask/1
  FDIR_Frame/13(nav_r_scale) -> Delay_nav_r_scale/1
  Delay_nav_mask/1 -> nav_mask/1
  Delay_nav_r_scale/1 -> nav_r_scale/1
  Table_tgrid/1 -> LQR_Low_Bandwidth/3
  Table_Target_Trajectory/1 -> LQR_Low_Bandwidth/4
  Table_K1flat_lo/1 -> LQR_Low_Bandwidth/5
  Table_K2grid/1 -> LQR_Low_Bandwidth/6
  Table_unom/1 -> LQR_Low_Bandwidth/7
  FDIR_Frame/1(abort) -> Delay_abort/1, Log_fdir_abort/1
  FDIR_Frame/2(safed) -> Delay_safed/1, Log_fdir_safed/1
  FDIR_Frame/3(degrade) -> Delay_degrade/1, Log_fdir_degrade/1
  FDIR_Frame/4(x_ref) -> Delay_x_ref/1
  FDIR_Frame/10(nav_abort) -> Delay_nav_abort/1
  LQR_Low_Bandwidth/1 -> Command_Select/2(u_lo)
  Delay_x_ref/1 -> Command_Select/4(x_ref)
  Delay_abort/1 -> Command_Select/6(abort)
  Delay_safed/1 -> Command_Select/7(safed)
  Delay_degrade/1 -> Command_Select/8(degrade)
  Delay_nav_abort/1 -> Command_Select/9(nav_abort)
  x_vert/1 -> Command_Select/10(x_vert)
  Command_Select/1(u) -> u/1, Delay_u_cmd/1
  Delay_u_cmd/1 -> FDIR_Frame/11(u_cmd)
  FDIR_Frame/5(mode) -> Log_fdir_mode/1
  FDIR_Frame/6(level) -> Log_fdir_level/1
  FDIR_Frame/7(first_fault) -> Log_fdir_first_fault/1
  FDIR_Frame/8(status) -> Log_fdir_status/1
  FDIR_Frame/9(raw) -> Log_fdir_raw/1
  FDIR_Frame/11(nav_nis) -> Log_fdir_nav_nis/1

== system hopper_6dof/Logging/Scopes_actuation/On ==
  act_bus : Inport
  gnc_bus : Inport  Port=2
  actuation : Scope  NumInputPorts=4
      settings: ActiveDisplayString=4  Title=Controller command u
  mux : Mux  Inputs=2
  sel_act_bus : BusSelector  OutputSignals=tvc_pitch,tvc_yaw,force,moment
  sel_gnc_bus : BusSelector  OutputSignals=u_cmd
  wires:
  sel_gnc_bus/1 -> actuation/4  "<u_cmd>"
  gnc_bus/1 -> sel_gnc_bus/1
  sel_act_bus/3 -> actuation/2  "<force>"
  sel_act_bus/1 -> mux/1  "<tvc_pitch>"
  act_bus/1 -> sel_act_bus/1
  sel_act_bus/4 -> actuation/3  "<moment>"
  sel_act_bus/2 -> mux/2  "<tvc_yaw>"
  mux/1 -> actuation/1

== system hopper_6dof/Logging/Scopes_attitude/On ==
  dyn_bus : Inport
  Gain : Gain  Gain=-1
  Gain1 : Gain  Gain=180/pi
  Gain2 : Gain  Gain=180/pi
  Reshape : Reshape
  Saturation : Saturate  UpperLimit=1  LowerLimit=-1
  Selector : Selector  InputPortWidth=9  IndexOptions=Index vector (dialog)  Indices=7  OutputSizes=1
  Trigonometric Function : Trigonometry  Operator=acos
  attitude : Scope  NumInputPorts=3
      settings: ActiveDisplayString=3  Title=Quaternion  ActiveDisplayYMinimum=-0.093579008937761818  ActiveDisplayYMaximum=0.80742680664889943
  sel_dyn_bus : BusSelector  OutputSignals=dcm_be,w_body,quat
  wires:
  sel_dyn_bus/2 -> Gain2/1  "<w_body>"
  dyn_bus/1 -> sel_dyn_bus/1
  sel_dyn_bus/3 -> attitude/3  "<quat>"
  sel_dyn_bus/1 -> Reshape/1  "<dcm_be>"
  Saturation/1 -> Gain/1
  Gain1/1 -> attitude/1  "dcm_be_tilt"
  Reshape/1 -> Selector/1
  Gain/1 -> Trigonometric Function/1
  Gain2/1 -> attitude/2  "w_body_deg"
  Selector/1 -> Saturation/1
  Trigonometric Function/1 -> Gain1/1

== system hopper_6dof/Logging/Scopes_environment/On ==
  env_bus : Inport
  environment : Scope  NumInputPorts=3
      settings: ActiveDisplayString=3  Title=Roll disturbance (N m)
  sel_env_bus : BusSelector  OutputSignals=wind_force,wind_moment,roll_dist
  wires:
  env_bus/1 -> sel_env_bus/1
  sel_env_bus/3 -> environment/3  "<roll_dist>"
  sel_env_bus/1 -> environment/1  "<wind_force>"
  sel_env_bus/2 -> environment/2  "<wind_moment>"

== system hopper_6dof/Logging/Scopes_fdir/On ==
  gnc_bus : Inport
  nav_bus : Inport  Port=2
  fdir : Scope  NumInputPorts=3
      settings: ActiveDisplayString=3  Title=Sensor valid flags
  sel_gnc_bus : BusSelector  OutputSignals=nav_mask,nav_r_scale
  sel_nav_bus : BusSelector  OutputSignals=valid
  wires:
  gnc_bus/1 -> sel_gnc_bus/1
  nav_bus/1 -> sel_nav_bus/1
  sel_nav_bus/1 -> fdir/3  "<valid>"
  sel_gnc_bus/1 -> fdir/1  "<nav_mask>"
  sel_gnc_bus/2 -> fdir/2  "<nav_r_scale>"

== system hopper_6dof/Logging/Scopes_mass_props/On ==
  prop_bus : Inport
  Reshape : Reshape
  Reshape1 : Reshape
  Selector : Selector  InputPortWidth=9  IndexOptions=Index vector (dialog)  Indices=[1 5 9]  OutputSizes=1
  Selector1 : Selector  InputPortWidth=9  IndexOptions=Index vector (dialog)  Indices=[1 5 9]  OutputSizes=1
  mass_props : Scope  NumInputPorts=5
      settings: ActiveDisplayString=5  Title=dI/dt diagonal (kg m^2/s)
  sel_prop_bus : BusSelector  OutputSignals=cg,cg_slosh,engine_cg,moi,moi_dot
  wires:
  Reshape1/1 -> Selector1/1
  sel_prop_bus/5 -> Reshape1/1  "<moi_dot>"
  sel_prop_bus/3 -> mass_props/3  "<engine_cg>"
  sel_prop_bus/1 -> mass_props/1  "<cg>"
  prop_bus/1 -> sel_prop_bus/1
  Reshape/1 -> Selector/1
  sel_prop_bus/4 -> Reshape/1  "<moi>"
  sel_prop_bus/2 -> mass_props/2  "<cg_slosh>"
  Selector/1 -> mass_props/4  "moi_diag"
  Selector1/1 -> mass_props/5  "moi_dot_diag"

== system hopper_6dof/Logging/Scopes_nav_attitude/On ==
  nav_bus : Inport
  dyn_bus : Inport  Port=2
  Gain : Gain  Gain=180/pi
  Gain1 : Gain  Gain=180/pi
  Selector : Selector  IndexOptions=Index vector (dialog)  Indices=[7:9]  OutputSizes=1
  Selector1 : Selector  IndexOptions=Index vector (dialog)  Indices=[10:13]  OutputSizes=1
  mux : Mux  Inputs=2
  mux1 : Mux  Inputs=2
  nav_attitude : Scope  NumInputPorts=2
      settings: Title=Quaternion: estimate vs truth  ActiveDisplayYMinimum=-0.11617755232450144  ActiveDisplayYMaximum=0.80993775591409267
  sel_dyn_bus : BusSelector  OutputSignals=w_body,quat
  sel_nav_bus : BusSelector  OutputSignals=x_nav
  wires:
  sel_dyn_bus/1 -> Gain1/1  "<w_body>"
  Gain/1 -> mux/1  "x_nav_7_9_deg"
  Selector/1 -> Gain/1
  dyn_bus/1 -> sel_dyn_bus/1
  nav_bus/1 -> sel_nav_bus/1
  sel_nav_bus/1 -> Selector1/1, Selector/1  "<x_nav>"
  sel_dyn_bus/2 -> mux1/2  "<quat>"
  Selector1/1 -> mux1/1  "x_nav_10_13"
  Gain1/1 -> mux/2  "w_body_deg"
  mux1/1 -> nav_attitude/2
  mux/1 -> nav_attitude/1

== system hopper_6dof/Logging/Scopes_navigation/On ==
  nav_bus : Inport
  dyn_bus : Inport  Port=2
  Selector : Selector  IndexOptions=Index vector (dialog)  Indices=[1:3]  OutputSizes=1
  Selector1 : Selector  IndexOptions=Index vector (dialog)  Indices=[4:6]  OutputSizes=1
  mux : Mux  Inputs=2
  mux1 : Mux  Inputs=2
  navigation : Scope  NumInputPorts=4
      settings: ActiveDisplayString=4  Title=Shadow estimator  ActiveDisplayYMinimum=-5.2180147694904662  ActiveDisplayYMaximum=2.0784764996978855
  sel_dyn_bus : BusSelector  OutputSignals=pos_ned,vel_ned
  sel_nav_bus : BusSelector  OutputSignals=x_nav,nav_diag,shadow
  wires:
  sel_nav_bus/1 -> Selector/1, Selector1/1  "<x_nav>"
  nav_bus/1 -> sel_nav_bus/1
  sel_nav_bus/2 -> navigation/3  "<nav_diag>"
  sel_dyn_bus/1 -> mux/2  "<pos_ned>"
  dyn_bus/1 -> sel_dyn_bus/1
  sel_nav_bus/3 -> navigation/4  "<shadow>"
  sel_dyn_bus/2 -> mux1/2  "<vel_ned>"
  Selector/1 -> mux/1  "x_nav_1_3"
  Selector1/1 -> mux1/1  "x_nav_4_6"
  mux/1 -> navigation/1
  mux1/1 -> navigation/2

== system hopper_6dof/Logging/Scopes_propulsion/On ==
  prop_bus : Inport
  act_bus : Inport  Port=2
  T_ts : FromWorkspace  VariableName=T_ts
  mux : Mux
  mux1 : Mux  Inputs=2
  propulsion : Scope  NumInputPorts=3
      settings: ActiveDisplayString=3  Title=Vehicle mass (kg)
  sel_act_bus : BusSelector  OutputSignals=thrust_cmd,thrust_req
  sel_prop_bus : BusSelector  OutputSignals=thrust,ox_mass,fu_mass,mass
  wires:
  prop_bus/1 -> sel_prop_bus/1
  sel_act_bus/1 -> mux/2  "<thrust_cmd>"
  sel_prop_bus/3 -> mux1/2  "<fu_mass>"
  T_ts/1 -> mux/4  "T_ts"
  act_bus/1 -> sel_act_bus/1
  sel_act_bus/2 -> mux/3  "<thrust_req>"
  sel_prop_bus/1 -> mux/1  "<thrust>"
  sel_prop_bus/2 -> mux1/1  "<ox_mass>"
  sel_prop_bus/4 -> propulsion/3  "<mass>"
  mux/1 -> propulsion/1
  mux1/1 -> propulsion/2
